simulink model "ResLoad_Rob"  (R2024b)
settings: Solver=ode5  StartTime=0.0  StopTime=3  FixedStep=1e-03  RelTol=1e-3
undefined symbols (not defined in the file): delta_n, DiscIntNeverNeededParam, K_rob, Ki_rob, National_Instruments, Nu, Nx, PCI, rads2rpm, rpm2rads, sens, T_sim, wc, wc2
libraries: sldrtlib x3, simulink x1
settings Model: SimulationMode=external  ExtModeTrigDuration=45001  Creator=lenovo  LastModifiedBy=aboulenien
settings DataIOCC: ReturnWorkspaceOutputs=off
settings HardwareCC: ProdBitPerLong=64  ProdHWDeviceType=Intel->x86-64 (Linux 64)
settings RTWCC: Description=Simulink Desktop Real-Time  SystemTargetFile=sldrt.tlc  TemplateMakefile=sldrt.tmf  RTWCompilerOptimization=on
settings CodeAppCC: MaxIdLength=95
settings SimulinkDesktopRealTimeCC: TargetLibSuffix=_sldrt.a  TargetPreCompLibLocation=C:\Program Files\MATLAB\R2024b\toolbox\sldrt\lib\win64  ParMdlRefBuildCompliant=on

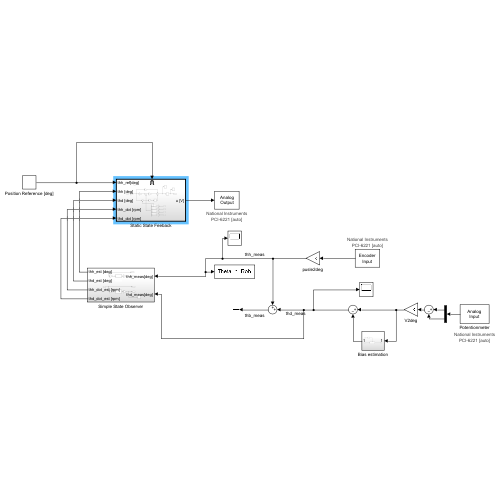
[thumbnail: Simulink's stored preview of the top-level diagram]
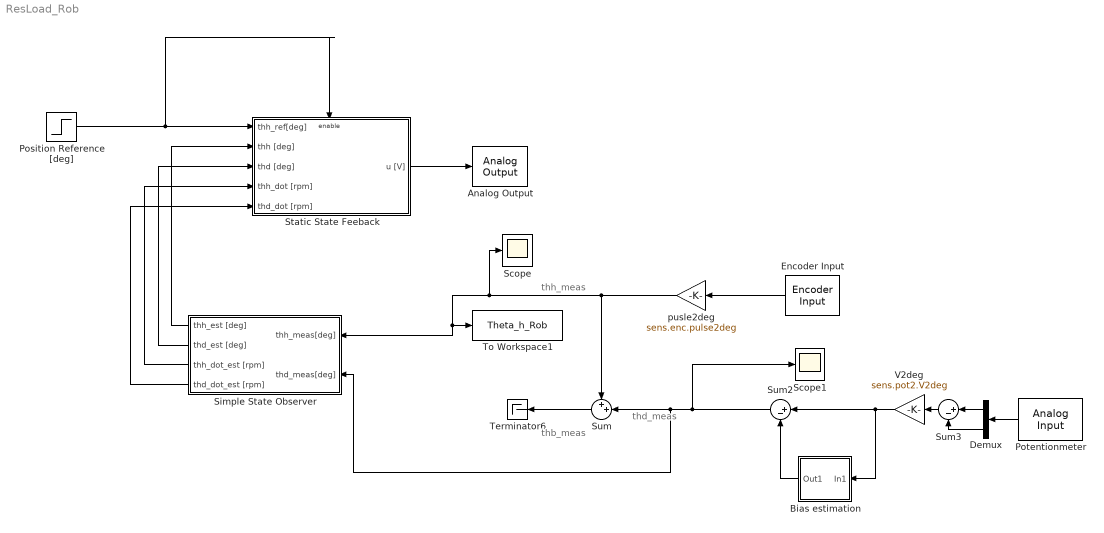
== system ResLoad_Rob ==
  note: thh_meas
  note: thb_meas
  note: thd_meas
  Analog Output : sldrtlib/Analog Output  SampleTime=-1  MaxMissedTicks=10  ShowMissedTicks=off  YieldWhenWaiting=off  DrvName=National_Instruments/PCI-6221  DrvAddress=4294967295  DrvOptions=[0 0 0 2 0]  Channels=1  RangeMode=1  VoltRange=1  InitialValue=0  FinalValue=0
      settings: AttributesFormatString=National Instruments\nPCI-6221 [auto]
  Bias estimation : Subsystem
  Demux : Demux  Outputs=2
  Encoder Input : sldrtlib/Encoder Input  SampleTime=T_sim  MaxMissedTicks=10  ShowMissedTicks=off  YieldWhenWaiting=off  DrvName=National_Instruments/PCI-6221  DrvAddress=4294967295  DrvOptions=[0 0 0 2 0]  Channels=1  QuadMode=3  IndexPulse=1  InputFilter=Inf  DataType=1
      settings: AttributesFormatString=National Instruments\nPCI-6221 [auto]
  Position Reference [deg] : Step  After=50  SampleTime=0
  Potentionmeter : sldrtlib/Analog Input  SampleTime=0.1  MaxMissedTicks=10  ShowMissedTicks=off  YieldWhenWaiting=off  DrvName=National_Instruments/PCI-6221  DrvAddress=4294967295  DrvOptions=[0 0 0 2 0]  Channels=[3 4]  RangeMode=1  VoltRange=2  DataType=1
      settings: AttributesFormatString=National Instruments\nPCI-6221 [auto]
  Scope : Scope
  Scope1 : Scope
  Simple State Observer : Subsystem
  Static State Feeback : Subsystem
  Sum : Sum  Inputs=++|
  Sum2 : Sum  Inputs=|+-
  Sum3 : Sum  Inputs=|+-
  Terminator6 : Terminator
  To Workspace1 : ToWorkspace  VariableName=Theta_h_Rob  SaveFormat=Structure With Time  SampleTime=0.001
  V2deg : Gain  Gain=sens.pot2.V2deg
  pusle2deg : Gain  Gain=sens.enc.pulse2deg
  wires:
  Sum2/1 -> Scope1/1, Simple State Observer/2(thd_meas[deg]), Sum/2
  pusle2deg/1 -> Simple State Observer/1(thh_meas[deg]), To Workspace1/1, Scope/1, Sum/1
  Sum/1 -> Terminator6/1
  Encoder Input/1 -> pusle2deg/1
  Bias estimation/1(Out1) -> Sum2/2
  Potentionmeter/1 -> Demux/1
  Demux/1 -> Sum3/1
  Demux/2 -> Sum3/2
  Sum3/1 -> V2deg/1
  V2deg/1 -> Bias estimation/1(In1), Sum2/1
  Simple State Observer/1(thh_est [deg]) -> Static State Feeback/2(thh [deg])
  Simple State Observer/2(thd_est [deg]) -> Static State Feeback/3(thd [deg])
  Simple State Observer/4(thd_dot_est [rpm]) -> Static State Feeback/5(thd_dot [rpm])
  Simple State Observer/3(thh_dot_est [rpm]) -> Static State Feeback/4(thh_dot [rpm])
  Static State Feeback/1(u [V]) -> Analog Output/1
  Position Reference [deg]/1 -> Static State Feeback/Enable, Static State Feeback/1(thh_ref[deg])

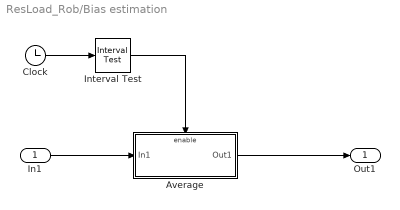
== system ResLoad_Rob/Bias estimation ==
  In1 : Inport
  Average : Subsystem  TreatAsAtomicUnit=on
  Clock : Clock
  Interval Test : simulink/Logic and Bit Operations/Interval Test  IntervalClosedRight=on  uplimit=0.7  IntervalClosedLeft=on  lowlimit=0.1  OutDataTypeStr=boolean
  Out1 : Outport
  wires:
  In1/1 -> Average/1(In1)
  Average/1(Out1) -> Out1/1
  Clock/1 -> Interval Test/1
  Interval Test/1 -> Average/Enable

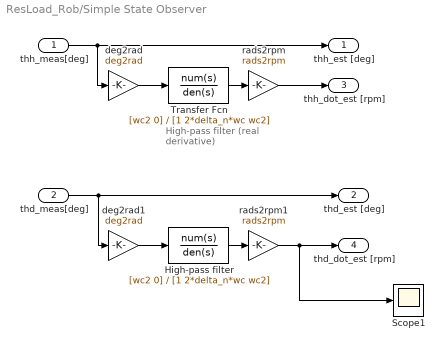
== system ResLoad_Rob/Simple State Observer ==
  note: High-pass filter
      | (real derivative)
  thh_meas[deg] : Inport
  thd_meas[deg] : Inport  Port=2
  "High-pass filter " : TransferFcn  Numerator=[wc2 0]  Denominator=[1 2*delta_n*wc wc2]
  Scope1 : Scope
  Transfer Fcn : TransferFcn  Numerator=[wc2 0]  Denominator=[1 2*delta_n*wc wc2]
  deg2rad : Gain  Gain=deg2rad
  deg2rad1 : Gain  Gain=deg2rad
  rads2rpm : Gain  Gain=rads2rpm
  rads2rpm1 : Gain  Gain=rads2rpm
  thh_est [deg] : Outport
  thd_est [deg] : Outport  Port=2
  thh_dot_est [rpm] : Outport  Port=3
  thd_dot_est [rpm] : Outport  Port=4
  wires:
  thh_meas[deg]/1 -> deg2rad/1, thh_est [deg]/1
  Transfer Fcn/1 -> rads2rpm/1
  thd_meas[deg]/1 -> thd_est [deg]/1, deg2rad1/1
  "High-pass filter "/1 -> rads2rpm1/1
  rads2rpm1/1 -> thd_dot_est [rpm]/1, Scope1/1
  deg2rad/1 -> Transfer Fcn/1
  deg2rad1/1 -> "High-pass filter "/1
  rads2rpm/1 -> thh_dot_est [rpm]/1

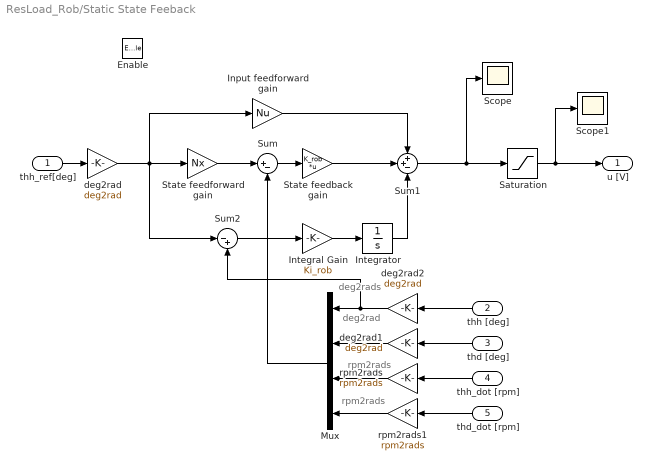
== system ResLoad_Rob/Static State Feeback ==
  note: deg2rads
  note: deg2rad
  note: rpm2rads
  note: rpm2rads
  thh_ref[deg] : Inport
  thh [deg] : Inport  Port=2
  thd [deg] : Inport  Port=3
  thh_dot [rpm] : Inport  Port=4
  thd_dot [rpm] : Inport  Port=5
  Enable : EnablePort
  Input feedforward gain : Gain  Gain=Nu
  Integral Gain : Gain  Gain=Ki_rob
  Integrator : Integrator
  Mux : Mux
  Saturation : Saturate  UpperLimit=12  LowerLimit=-12
  Scope : Scope
  Scope1 : Scope
  State feedback gain : Gain  Gain=K_rob  Multiplication=Matrix(K*u)
  State feedforward gain : Gain  Gain=Nx
  Sum : Sum  Inputs=|+-
  Sum1 : Sum  Inputs=++-
  Sum2 : Sum  Inputs=|-+
  deg2rad : Gain  Gain=deg2rad
  deg2rad1 : Gain  Gain=deg2rad
  deg2rad2 : Gain  Gain=deg2rad
  rpm2rads : Gain  Gain=rpm2rads
  rpm2rads1 : Gain  Gain=rpm2rads
  u [V] : Outport
  wires:
  thh_ref[deg]/1 -> deg2rad/1
  deg2rad/1 -> Sum2/1, State feedforward gain/1, Input feedforward gain/1
  State feedforward gain/1 -> Sum/1
  Sum/1 -> State feedback gain/1
  Saturation/1 -> Scope1/1, u [V]/1
  Mux/1 -> Sum/2
  deg2rad2/1 -> Sum2/2, Mux/1
  thh [deg]/1 -> deg2rad2/1
  Input feedforward gain/1 -> Sum1/1
  Sum1/1 -> Scope/1, Saturation/1
  State feedback gain/1 -> Sum1/2
  rpm2rads1/1 -> Mux/4
  Sum2/1 -> Integral Gain/1
  Integral Gain/1 -> Integrator/1
  Integrator/1 -> Sum1/3
  deg2rad1/1 -> Mux/2
  rpm2rads/1 -> Mux/3
  thd [deg]/1 -> deg2rad1/1
  thh_dot [rpm]/1 -> rpm2rads/1
  thd_dot [rpm]/1 -> rpm2rads1/1

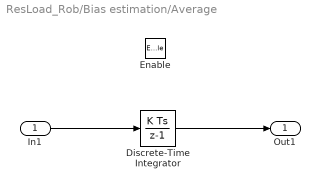
== system ResLoad_Rob/Bias estimation/Average ==
  In1 : Inport
  Enable : EnablePort
  Discrete-Time Integrator : DiscreteIntegrator  gainval=2  SampleTime=-1  ICPrevOutput=DiscIntNeverNeededParam  ICPrevScaledInput=DiscIntNeverNeededParam
  Out1 : Outport
  wires:
  In1/1 -> Discrete-Time Integrator/1
  Discrete-Time Integrator/1 -> Out1/1
